simulink model "SarBehavior.as_run"  (R2024a)
settings: Solver=VariableStepDiscrete  StartTime=0  StopTime=P.stop_time_s  RelTol=1e-3
model workspace (MAT data in the model file):
  DecodeP.schema = 'sar20-behavior-decode/v1'
  DecodeP.vref_v = 4.096
  DecodeP.fsr_diff_v = 8.192
  DecodeP.ra_gain = 32
  DecodeP.d2_weights_ra_v = [0.36; 0.24; 0.16; 0.104; 0.064; 0.04; 0.024; 0.012; 0.008; 0.004; 0.002; 0.001]
  DecodeP.d2_offset_ra_v = -0.5095
  DecodeP.tracking_step_ra_v = 0.00025
  DecodeP.dither_enabled = 0
  DecodeP.dither_seed = 20261223
  DecodeP.dither_amplitude_v = 0.001
  DecodeP.calibration_mode = 'off'
  DecodeP.tracking_mode = 'finite_sinc2'
  DecodeP.coefficient_source = 'nominal saved.fpga weights only; new DAC1 geometry formula'
  P : object (value not decoded)
symbols that are objects in the model workspace (value not decoded): P
settings Model: Creator=Administrator  LastModifiedBy=Administrator
settings DataIOCC: SignalLogging=off

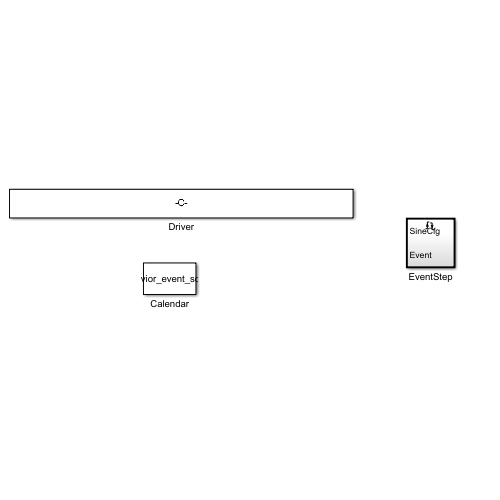
[thumbnail: Simulink's stored preview of the top-level diagram]
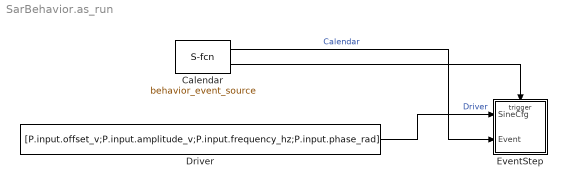
== system SarBehavior.as_run ==
  Calendar : M-S-Function  FunctionName=behavior_event_source  Parameters=P.schedule
  Driver : Constant  Value=[P.input.offset_v;P.input.amplitude_v;P.input.frequency_hz;P.input.phase_rad]
  EventStep : Subsystem
  wires:
  Calendar/1 -> EventStep/2(Event)  "Calendar"
  Driver/1 -> EventStep/1(SineCfg)  "Driver"
  Calendar/2 -> EventStep/Trigger

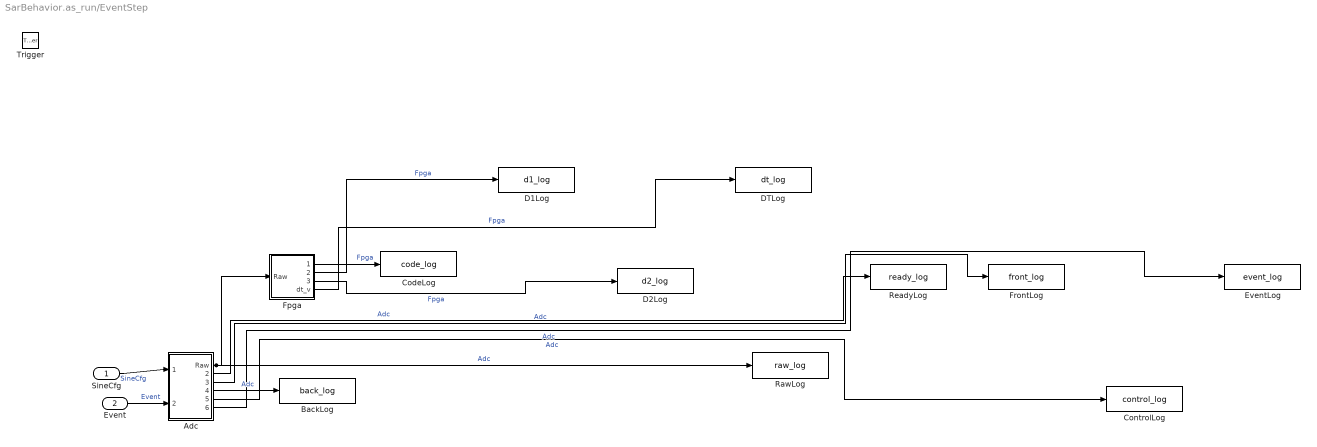
== system SarBehavior.as_run/EventStep ==
  SineCfg : Inport  PortDimensions=4
  Event : Inport  Port=2  PortDimensions=2
  Trigger : TriggerPort  TriggerType=either  VariantControl=(inherit)  ZeroCross=off  InitialTriggerSignalState=zero  PortDimensions=1
  Adc : Subsystem
  BackLog : ToWorkspace  VariableName=back_log  SaveFormat=Timeseries  SampleTime=-1
  CodeLog : ToWorkspace  VariableName=code_log  SaveFormat=Timeseries  SampleTime=-1
  ControlLog : ToWorkspace  VariableName=control_log  SaveFormat=Timeseries  SampleTime=-1
  D1Log : ToWorkspace  VariableName=d1_log  SaveFormat=Timeseries  SampleTime=-1
  D2Log : ToWorkspace  VariableName=d2_log  SaveFormat=Timeseries  SampleTime=-1
  DTLog : ToWorkspace  VariableName=dt_log  SaveFormat=Timeseries  SampleTime=-1
  EventLog : ToWorkspace  VariableName=event_log  SaveFormat=Timeseries  SampleTime=-1
  Fpga : Subsystem
  FrontLog : ToWorkspace  VariableName=front_log  SaveFormat=Timeseries  SampleTime=-1
  RawLog : ToWorkspace  VariableName=raw_log  SaveFormat=Timeseries  SampleTime=-1
  ReadyLog : ToWorkspace  VariableName=ready_log  SaveFormat=Timeseries  SampleTime=-1
  wires:
  Fpga/4(dt_v) -> DTLog/1  "Fpga"
  Fpga/3(d2_v) -> D2Log/1  "Fpga"
  Fpga/2(d1_v) -> D1Log/1  "Fpga"
  Fpga/1(code20) -> CodeLog/1  "Fpga"
  Adc/6(Event) -> EventLog/1  "Adc"
  Adc/5(Control) -> ControlLog/1  "Adc"
  Adc/4(Backend) -> BackLog/1  "Adc"
  Adc/3(Frontend) -> FrontLog/1  "Adc"
  Adc/2(Ready) -> ReadyLog/1  "Adc"
  Adc/1(Raw) -> RawLog/1, Fpga/1(Raw)  "Adc"
  Event/1 -> Adc/2(Calendar)  "Event"
  SineCfg/1 -> Adc/1(SineCfg)  "SineCfg"

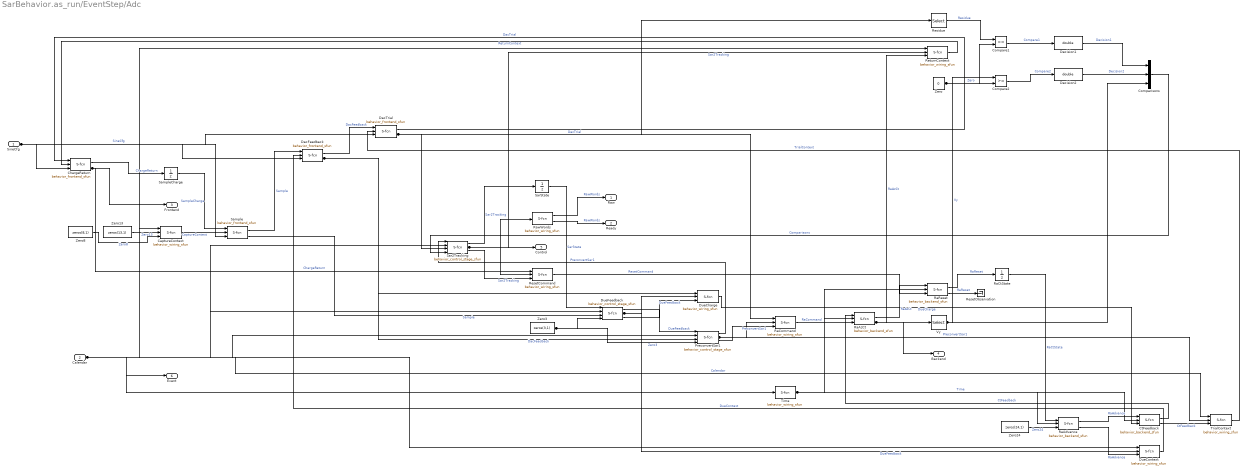
== system SarBehavior.as_run/EventStep/Adc ==
  SineCfg : Inport  PortDimensions=4
  Calendar : Inport  Port=2  PortDimensions=2
  CaptureContext : M-S-Function  FunctionName=behavior_wiring_sfun  Parameters='cnv',P
  ChargeReturn : M-S-Function  FunctionName=behavior_frontend_sfun  Parameters='commit',P.front
  Compare1 : RelationalOperator  OutDataTypeStr=boolean  RndMeth=Simplest  InputSameDT=off
  Compare2 : RelationalOperator  OutDataTypeStr=boolean  RndMeth=Simplest  InputSameDT=off
  Comparisons : Mux  Inputs=3
  CtFeedback : M-S-Function  FunctionName=behavior_backend_sfun  Parameters='commit',P.backend
  DacFeedback : M-S-Function  FunctionName=behavior_frontend_sfun  Parameters='commit',P.front
  DacTrial : M-S-Function  FunctionName=behavior_frontend_sfun  Parameters='commit',P.front
  Decision1 : DataTypeConversion  OutDataTypeStr=double  SaturateOnIntegerOverflow=off  RndMeth=Floor
  Decision2 : DataTypeConversion  OutDataTypeStr=double  SaturateOnIntegerOverflow=off  RndMeth=Floor
  DueCharge : M-S-Function  FunctionName=behavior_wiring_sfun  Parameters='backend',P
  DueContext : M-S-Function  FunctionName=behavior_wiring_sfun  Parameters='due',P
  DueFeedback : M-S-Function  FunctionName=behavior_control_stage_sfun  Parameters='due',P
  PreconvertSar1 : M-S-Function  FunctionName=behavior_control_stage_sfun  Parameters='prepare',P
  RaAdvance : M-S-Function  FunctionName=behavior_backend_sfun  Parameters='advance',P.backend
  RaAzCt : M-S-Function  FunctionName=behavior_backend_sfun  Parameters='commit',P.backend
  RaCommand : M-S-Function  FunctionName=behavior_wiring_sfun  Parameters='backend',P
  RaCtState : UnitDelay  InitialCondition=P.xBK0  SampleTime=-1  HasFrameUpgradeWarning=on
  RaReset : M-S-Function  FunctionName=behavior_backend_sfun  Parameters='commit',P.backend
  RawWords : M-S-Function  FunctionName=behavior_wiring_sfun  Parameters='raw',P
  ResetCommand : M-S-Function  FunctionName=behavior_wiring_sfun  Parameters='backend',P
  ResetObservation : Terminator
  Residue : Selector  InputPortWidth=7  IndexOptions=Index vector (dialog)  Indices=2  OutputSizes=1
  ReturnContext : M-S-Function  FunctionName=behavior_wiring_sfun  Parameters='release',P
  Sample : M-S-Function  FunctionName=behavior_frontend_sfun  Parameters='advance',P.front
  SampleCharge : UnitDelay  InitialCondition=P.xFE0  SampleTime=-1  HasFrameUpgradeWarning=on
  Sar2Tracking : M-S-Function  FunctionName=behavior_control_stage_sfun  Parameters='decide',P
  SarState : UnitDelay  InitialCondition=P.xSC0  SampleTime=-1  HasFrameUpgradeWarning=on
  Time : M-S-Function  FunctionName=behavior_wiring_sfun  Parameters='clock',P
  TrialContext : M-S-Function  FunctionName=behavior_wiring_sfun  Parameters='trial',P
  Vy : Selector  InputPortWidth=8  IndexOptions=Index vector (dialog)  Indices=2  OutputSizes=1
  Zero : Constant  Value=0
  Zero13 : Constant  Value=zeros(13,1)
  Zero24 : Constant  Value=zeros(24,1)
  Zero3 : Constant  Value=zeros(3,1)
  Zero8 : Constant  Value=zeros(8,1)
  Raw : Outport  PortDimensions=6
  Ready : Outport  Port=2  PortDimensions=1
  Frontend : Outport  Port=3  PortDimensions=7
  Backend : Outport  Port=4  PortDimensions=8
  Control : Outport  Port=5  PortDimensions=13
  Event : Outport  Port=6  PortDimensions=2
  wires:
  RaReset/2 -> ResetObservation/1  "RaReset"
  RawWords/2 -> Ready/1  "RawWords"
  RawWords/1 -> Raw/1  "RawWords"
  Sar2Tracking/1 -> SarState/1  "Sar2Tracking"
  RaReset/1 -> RaCtState/1  "RaReset"
  ChargeReturn/1 -> SampleCharge/1  "ChargeReturn"
  ResetCommand/1 -> RaReset/3  "ResetCommand"
  RaAzCt/1 -> RaReset/1  "RaAzCt"
  Sar2Tracking/3 -> ResetCommand/3  "Sar2Tracking"
  ChargeReturn/2 -> Frontend/1, ResetCommand/1  "ChargeReturn"
  ReturnContext/1 -> ChargeReturn/2  "ReturnContext"
  DacTrial/1 -> ChargeReturn/1  "DacTrial"
  Sar2Tracking/2 -> Control/1, RawWords/1, ResetCommand/2, ReturnContext/2  "Sar2Tracking"
  Comparisons/1 -> Sar2Tracking/4  "Comparisons"
  PreconvertSar1/1 -> Sar2Tracking/1  "PreconvertSar1"
  Decision2/1 -> Comparisons/2  "Decision2"
  Decision1/1 -> Comparisons/1  "Decision1"
  Compare2/1 -> Decision2/1  "Compare2"
  Vy/1 -> Comparisons/3, Compare2/1  "Vy"
  Compare1/1 -> Decision1/1  "Compare1"
  Zero/1 -> Compare2/2, Compare1/2  "Zero"
  Residue/1 -> Compare1/1  "Residue"
  RaAzCt/2 -> Backend/1, ReturnContext/3, Vy/1  "RaAzCt"
  RaCommand/1 -> RaAzCt/3  "RaCommand"
  CtFeedback/1 -> RaAzCt/1  "CtFeedback"
  PreconvertSar1/3 -> RaCommand/3  "PreconvertSar1"
  DacTrial/2 -> Sar2Tracking/3, Residue/1, RaCommand/1  "DacTrial"
  TrialContext/1 -> DacTrial/2  "TrialContext"
  DacFeedback/1 -> DacTrial/1  "DacFeedback"
  CtFeedback/2 -> TrialContext/3  "CtFeedback"
  PreconvertSar1/2 -> RaCommand/2, TrialContext/2  "PreconvertSar1"
  DueFeedback/1 -> PreconvertSar1/1  "DueFeedback"
  DueCharge/1 -> CtFeedback/3  "DueCharge"
  RaAdvance/1 -> CtFeedback/1  "RaAdvance"
  DueFeedback/3 -> DueCharge/3  "DueFeedback"
  DacFeedback/2 -> PreconvertSar1/3, DueCharge/1  "DacFeedback"
  DueContext/1 -> DacFeedback/2  "DueContext"
  Sample/1 -> DacFeedback/1  "Sample"
  RaAdvance/2 -> DueContext/3  "RaAdvance"
  DueFeedback/2 -> DueCharge/2, DueContext/2  "DueFeedback"
  Zero3/1 -> PreconvertSar1/4, DueFeedback/4  "Zero3"
  Sample/2 -> DueFeedback/3  "Sample"
  SarState/1 -> DueFeedback/1  "SarState"
  Zero24/1 -> RaAdvance/3  "Zero24"
  Time/1 -> RaReset/2, RaAzCt/2, CtFeedback/2, RaAdvance/2  "Time"
  RaCtState/1 -> RaAdvance/1  "RaCtState"
  SineCfg/1 -> ChargeReturn/3, DacTrial/3, DacFeedback/3, Sample/3  "SineCfg"
  CaptureContext/1 -> Sample/2  "CaptureContext"
  SampleCharge/1 -> Sample/1  "SampleCharge"
  Zero8/1 -> CaptureContext/3  "Zero8"
  Zero13/1 -> CaptureContext/2  "Zero13"
  Calendar/1 -> Event/1, ReturnContext/1, Sar2Tracking/2, TrialContext/1, PreconvertSar1/2, DueContext/1, DueFeedback/2, CaptureContext/1, Time/1  "Calendar"

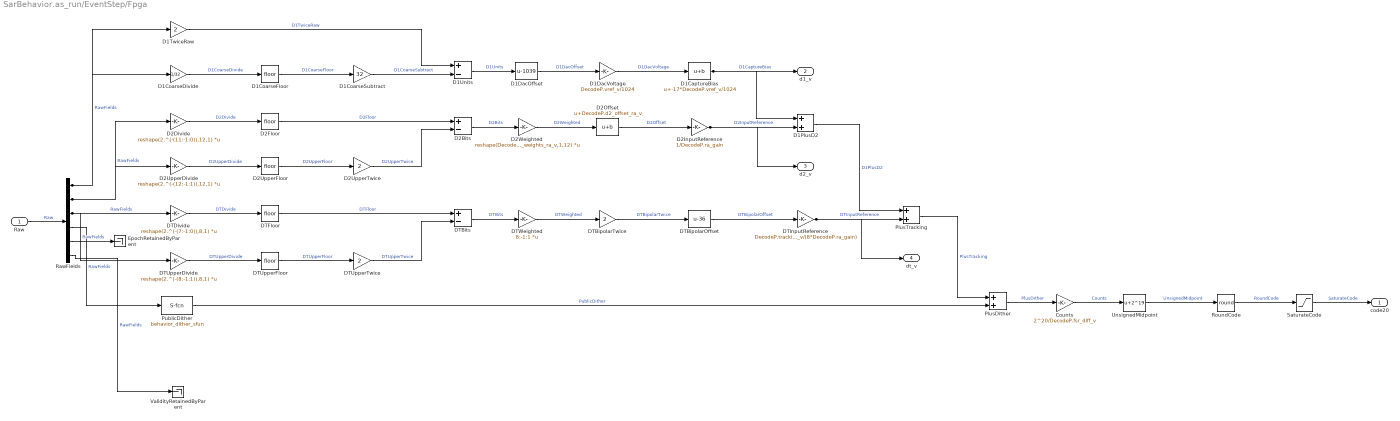
== system SarBehavior.as_run/EventStep/Fpga ==
  Raw : Inport  PortDimensions=6
  Counts : Gain  Gain=2^20/DecodeP.fsr_diff_v
  D1CaptureBias : Bias  Bias=-17*DecodeP.vref_v/1024  SaturateOnIntegerOverflow=off
  D1CoarseDivide : Gain  Gain=1/32
  D1CoarseFloor : Rounding
  D1CoarseSubtract : Gain  Gain=32
  D1DacOffset : Bias  Bias=-1039  SaturateOnIntegerOverflow=off
  D1DacVoltage : Gain  Gain=DecodeP.vref_v/1024
  D1PlusD2 : Sum
  D1TwiceRaw : Gain  Gain=2
  D1Units : Sum  Inputs=+-
  D2Bits : Sum  Inputs=+-
  D2Divide : Gain  Gain=reshape(2.^(-(11:-1:0)),12,1)  Multiplication=Matrix(K*u)
  D2Floor : Rounding
  D2InputReference : Gain  Gain=1/DecodeP.ra_gain
  D2Offset : Bias  Bias=DecodeP.d2_offset_ra_v  SaturateOnIntegerOverflow=off
  D2UpperDivide : Gain  Gain=reshape(2.^(-(12:-1:1)),12,1)  Multiplication=Matrix(K*u)
  D2UpperFloor : Rounding
  D2UpperTwice : Gain  Gain=2
  D2Weighted : Gain  Gain=reshape(DecodeP.d2_weights_ra_v,1,12)  Multiplication=Matrix(K*u)
  DTBipolarOffset : Bias  Bias=-36  SaturateOnIntegerOverflow=off
  DTBipolarTwice : Gain  Gain=2
  DTBits : Sum  Inputs=+-
  DTDivide : Gain  Gain=reshape(2.^(-(7:-1:0)),8,1)  Multiplication=Matrix(K*u)
  DTFloor : Rounding
  DTInputReference : Gain  Gain=DecodeP.tracking_step_ra_v/(8*DecodeP.ra_gain)
  DTUpperDivide : Gain  Gain=reshape(2.^(-(8:-1:1)),8,1)  Multiplication=Matrix(K*u)
  DTUpperFloor : Rounding
  DTUpperTwice : Gain  Gain=2
  DTWeighted : Gain  Gain=8:-1:1  Multiplication=Matrix(K*u)
  EpochRetainedByParent : Terminator
  PlusDither : Sum
  PlusTracking : Sum
  PublicDither : M-S-Function  FunctionName=behavior_dither_sfun  Parameters=DecodeP
  RawFields : Demux  Outputs=6
  RoundCode : Rounding  Operator=round
  SaturateCode : Saturate  UpperLimit=2^20-1  LowerLimit=0
  UnsignedMidpoint : Bias  Bias=2^19  SaturateOnIntegerOverflow=off
  ValidityRetainedByParent : Terminator
  code20 : Outport  PortDimensions=1
  d1_v : Outport  Port=2  PortDimensions=1
  d2_v : Outport  Port=3  PortDimensions=1
  dt_v : Outport  Port=4  PortDimensions=1
  wires:
  DTUpperTwice/1 -> DTBits/2  "DTUpperTwice"
  DTFloor/1 -> DTBits/1  "DTFloor"
  DTUpperFloor/1 -> DTUpperTwice/1  "DTUpperFloor"
  DTUpperDivide/1 -> DTUpperFloor/1  "DTUpperDivide"
  DTDivide/1 -> DTFloor/1  "DTDivide"
  RawFields/3 -> DTUpperDivide/1, DTDivide/1  "RawFields"
  D2UpperTwice/1 -> D2Bits/2  "D2UpperTwice"
  D2Floor/1 -> D2Bits/1  "D2Floor"
  D2UpperFloor/1 -> D2UpperTwice/1  "D2UpperFloor"
  D2UpperDivide/1 -> D2UpperFloor/1  "D2UpperDivide"
  D2Divide/1 -> D2Floor/1  "D2Divide"
  RawFields/2 -> D2UpperDivide/1, D2Divide/1  "RawFields"
  SaturateCode/1 -> code20/1  "SaturateCode"
  RoundCode/1 -> SaturateCode/1  "RoundCode"
  UnsignedMidpoint/1 -> RoundCode/1  "UnsignedMidpoint"
  Counts/1 -> UnsignedMidpoint/1  "Counts"
  PlusDither/1 -> Counts/1  "PlusDither"
  PublicDither/1 -> PlusDither/2  "PublicDither"
  PlusTracking/1 -> PlusDither/1  "PlusTracking"
  DTInputReference/1 -> dt_v/1, PlusTracking/2  "DTInputReference"
  D1PlusD2/1 -> PlusTracking/1  "D1PlusD2"
  D2InputReference/1 -> d2_v/1, D1PlusD2/2  "D2InputReference"
  D1CaptureBias/1 -> d1_v/1, D1PlusD2/1  "D1CaptureBias"
  RawFields/6 -> ValidityRetainedByParent/1  "RawFields"
  RawFields/5 -> EpochRetainedByParent/1  "RawFields"
  RawFields/4 -> PublicDither/1  "RawFields"
  DTBipolarOffset/1 -> DTInputReference/1  "DTBipolarOffset"
  DTBipolarTwice/1 -> DTBipolarOffset/1  "DTBipolarTwice"
  DTWeighted/1 -> DTBipolarTwice/1  "DTWeighted"
  DTBits/1 -> DTWeighted/1  "DTBits"
  D2Offset/1 -> D2InputReference/1  "D2Offset"
  D2Weighted/1 -> D2Offset/1  "D2Weighted"
  D2Bits/1 -> D2Weighted/1  "D2Bits"
  D1DacVoltage/1 -> D1CaptureBias/1  "D1DacVoltage"
  D1DacOffset/1 -> D1DacVoltage/1  "D1DacOffset"
  D1Units/1 -> D1DacOffset/1  "D1Units"
  D1CoarseSubtract/1 -> D1Units/2  "D1CoarseSubtract"
  D1TwiceRaw/1 -> D1Units/1  "D1TwiceRaw"
  D1CoarseFloor/1 -> D1CoarseSubtract/1  "D1CoarseFloor"
  D1CoarseDivide/1 -> D1CoarseFloor/1  "D1CoarseDivide"
  RawFields/1 -> D1TwiceRaw/1, D1CoarseDivide/1  "RawFields"
  Raw/1 -> RawFields/1  "Raw"
